simulink model "DMC_FCSMPC_IM_Physical_v6_3_L100_T1_EX28"  (R2021a)
settings: Solver=FixedStepDiscrete  StartTime=0.0  StopTime=3  FixedStep=1e-6  RelTol=1e-3
libraries: spsIGBTDiodeLib x18, spsCurrentMeasurementLib x3, spsThreePhaseSeriesRLCBranchLib x3, spsThreePhaseVIMeasurementLib x3, spsThreePhaseParallelRLCBranchLib x2, spsAsynchronousMachineSIUnitsLib x1, spsThreePhaseProgrammableVoltageSourceLib x1, spsGroundLib x1, spspowerguiLib x1
settings Model: Creator=edula  LastModifiedBy=Usuario

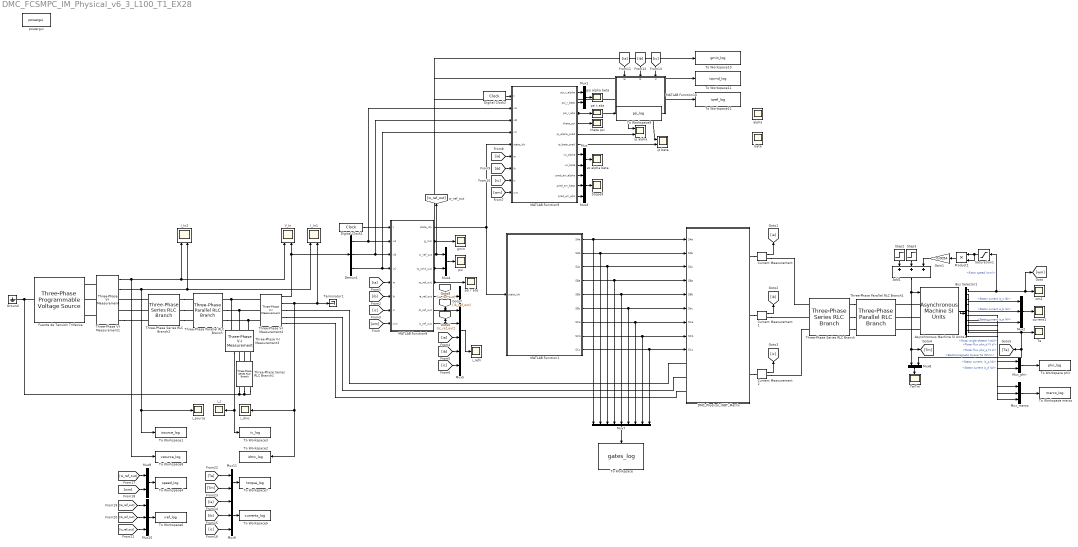
== system DMC_FCSMPC_IM_Physical_v6_3_L100_T1_EX28 ==
  Add1 : Sum  Inputs=+++
  Asynchronous Machine SI Units1 : spsAsynchronousMachineSIUnitsLib/Asynchronous Machine SI Units  RotorType=Squirrel-cage  PresetModel=No  MechanicalLoad=Torque Tm  ShowDetailedParameters=on  ReferenceFrame=Rotor  Units=SI  MeasurementBus=off  NominalParameters=[1.845e+04 380 50]  VoltageRatio=1  Stator=[0.5968 0.0003495]  Rotor=[0.6258 0.005473]  Cage1=[0.4155 0.002066]  Cage2=[0.4168 0.0003495]  Lm=0.0354  Mechanical=[0.08 0.005879 2]  PolePairs=2  InitialConditions=[1 0 0 0 0 0 0 0]  SimulateSaturation=off  Saturation=[14.03593122, 27.81365428, 53.79336849, 72.68890987, 97.98006896, 148.6815601, 215.7428561, 302.9841135, 428.7778367 ; 230, 322, 414, 460, 506, 552, 598, 644, 690]  LoadFlowParameters=1492000  TsPowergui=0  TsBlock=-1  IterativeModel=Trapezoidal non iterative  IterativeDiscreteModel=Trapezoidal non iterative  Pmec=1.492e+006
  Bus Selector1 : BusSelector  OutputSignals="Mechanical.Rotor speed (wm),Stator measurements.Stator current is_c (A),Stator measurements.Stator current is_b (A),Stator measurements.Stator current is_a (A),Mechanical.Electromagnetic torque Te (N*m),Rotor measurements.Rotor flux phir_q (V s),Rotor measurements.Rotor flux phir_d (V s),Mechanical.Rotor angle thetam (rad),Stator measurements.Stator current  is_q (A),Stator measurements.Stator current is_d (A)"
  Current Measurement : spsCurrentMeasurementLib/Current Measurement  PhasorSimulation=off  OutputType=Complex  PSBequivalent=0
  Current Measurement1 : spsCurrentMeasurementLib/Current Measurement  PhasorSimulation=off  OutputType=Complex  PSBequivalent=0
  Current Measurement2 : spsCurrentMeasurementLib/Current Measurement  PhasorSimulation=off  OutputType=Complex  PSBequivalent=0
  DMC_Physical_IGBT_Matrix : Subsystem
  Demux1 : Demux  Outputs=3
  Digital Clock1 : DigitalClock  SampleTime=1e-06
  Digital Clock2 : DigitalClock  SampleTime=1e-06
  Fuente de Tensión Trifásica : spsThreePhaseProgrammableVoltageSourceLib/Three-Phase Programmable Voltage Source  PositiveSequence=[380 0 50]  VariationEntity=Frequency  VariationType=Step  VariationTypeAlt=Ramp  VariationStep=0.5  VariationRate=0  VariationMagnitude=0.3  VariationFrequency=2  VariationTiming=[2 4]  VariationPhaseA=off  Amplitudes=[1 0.8 1.2 1.0]  TimeValues=[0 0.1 0.15 0.2]  HarmonicGeneration=off  HarmonicA=[3 0.2 -25 0]  HarmonicB=[2 0.15 35 2]  Timing="[0.05  3]"  BusType=swing  Pref=0  Qref=0  Qmin=-inf  Qmax=inf
  Gain1 : Gain  Gain=0.0054
  Ground : spsGroundLib/Ground  LConnTagsString=a
  I_In1 : Scope  NumInputPorts=2
  I_In2 : Scope  NumInputPorts=2
  MATLAB Function1 : MATLAB Function  TreatAsAtomicUnit=on
  MATLAB Function10 : MATLAB Function  TreatAsAtomicUnit=on
  MATLAB Function8 : MATLAB Function  TreatAsAtomicUnit=on
  MATLAB Function9 : MATLAB Function  TreatAsAtomicUnit=on
  Mux{,1,4,8..9,11} (6 alike) : Mux  Inputs=2
  Mux{2..3,6,10} (4 alike) : Mux  Inputs=3
  Mux5 : Mux  Inputs=6
  Mux7 : Mux  Inputs=9
  Mux_marco : Mux  Inputs=3
  Mux_phir : Mux  Inputs=2
  Product1 : Product  RndMeth=Zero
  Saturation1 : Saturate  UpperLimit=100000  LowerLimit=0
  Scope9 : Scope
  Step2 : Step  Time=0  After=0  SampleTime=0
  Step3 : Step  Time=0  After=5  SampleTime=0
  Te : Scope
  Te/Tm : Scope
  Terminator1 : Terminator
  Three-Phase Parallel RLC Branch : spsThreePhaseParallelRLCBranchLib/Three-Phase Parallel RLC Branch  LConnTagsString=A|B|C  RConnTagsString=A|B|C  BranchType=RL  Resistance=10  Inductance=0.0023  Capacitance=1.0  Measurements=None
      settings: SourceProductBaseCode=PS
  Three-Phase Parallel RLC Branch1 : spsThreePhaseParallelRLCBranchLib/Three-Phase Parallel RLC Branch  LConnTagsString=A|B|C  RConnTagsString=A|B|C  BranchType=RL  Resistance=25  Inductance=0.00000795  Capacitance=1e-6  Measurements=None
      settings: SourceProductBaseCode=PS
  Three-Phase Series RLC Branch : spsThreePhaseSeriesRLCBranchLib/Three-Phase Series RLC Branch  LConnTagsString=A|B|C  RConnTagsString=A|B|C  BranchType=R  Resistance=0.0525  Inductance=1e-3  Capacitance=1e-6  Measurements=None
  Three-Phase Series RLC Branch1 : spsThreePhaseSeriesRLCBranchLib/Three-Phase Series RLC Branch  LConnTagsString=A|B|C  RConnTagsString=A|B|C  BranchType=C  Resistance=1.0  Inductance=1.0  Capacitance=0.00001  Measurements=None
  Three-Phase Series RLC Branch2 : spsThreePhaseSeriesRLCBranchLib/Three-Phase Series RLC Branch  LConnTagsString=A|B|C  RConnTagsString=A|B|C  BranchType=RL  Resistance=0.0134  Inductance=0.0000259  Capacitance=1.0  Measurements=None
  Three-Phase V-I Measurement1 : spsThreePhaseVIMeasurementLib/Three-Phase V-I Measurement  VoltageMeasurement=phase-to-ground  SetLabelV=off  LabelV=Vabc  Vpu=off  VpuLL=off  CurrentMeasurement=yes  SetLabelI=off  LabelI=Iabc  Ipu=off  Pbase=100e6  Vbase=500e3  OutputType=Complex  PhasorSimulation=off  PSBequivalent=0
  Three-Phase V-I Measurement2 : spsThreePhaseVIMeasurementLib/Three-Phase V-I Measurement  VoltageMeasurement=phase-to-ground  SetLabelV=off  LabelV=Vabc  Vpu=off  VpuLL=off  CurrentMeasurement=yes  SetLabelI=off  LabelI=Iabc  Ipu=off  Pbase=100e6  Vbase=500e3  OutputType=Complex  PhasorSimulation=off  PSBequivalent=0
  Three-Phase V-I Measurement3 : spsThreePhaseVIMeasurementLib/Three-Phase V-I Measurement  VoltageMeasurement=phase-to-ground  SetLabelV=off  LabelV=Vabc  Vpu=off  VpuLL=off  CurrentMeasurement=yes  SetLabelI=off  LabelI=Iabc  Ipu=off  Pbase=100e6  Vbase=500e3  OutputType=Complex  PhasorSimulation=off  PSBequivalent=0
  To Workspace : ToWorkspace  VariableName=gates_log  SaveFormat=Structure With Time  SampleTime=-1
      settings: Decimation=200
  To Workspace marco : ToWorkspace  VariableName=marco_log  SaveFormat=Structure With Time  SampleTime=-1
      settings: Decimation=200
  To Workspace phir : ToWorkspace  VariableName=phir_log  SaveFormat=Structure With Time  SampleTime=-1
      settings: Decimation=200
  To Workspace1 : ToWorkspace  VariableName=isource_log  SaveFormat=Structure With Time  SampleTime=-1
      settings: Decimation=200
  To Workspace10 : ToWorkspace  VariableName=gmin_log  SaveFormat=Structure With Time  SampleTime=-1
      settings: Decimation=200
  To Workspace11 : ToWorkspace  VariableName=iqcmd_log  SaveFormat=Structure With Time  SampleTime=-1
      settings: Decimation=200
  To Workspace12 : ToWorkspace  VariableName=iqref_log  SaveFormat=Structure With Time  SampleTime=-1
      settings: Decimation=200
  To Workspace2 : ToWorkspace  VariableName=idmc_log  SaveFormat=Structure With Time  SampleTime=-1
      settings: Decimation=200
  To Workspace3 : ToWorkspace  VariableName=ic_log  SaveFormat=Structure With Time  SampleTime=-1
      settings: Decimation=200
  To Workspace4 : ToWorkspace  VariableName=speed_log  SaveFormat=Structure With Time  SampleTime=-1
      settings: Decimation=200
  To Workspace5 : ToWorkspace  VariableName=currents_log  SaveFormat=Structure With Time  SampleTime=-1
      settings: Decimation=200
  To Workspace6 : ToWorkspace  VariableName=iref_log  SaveFormat=Structure With Time  SampleTime=-1
      settings: Decimation=200
  To Workspace7 : ToWorkspace  VariableName=torque_log  SaveFormat=Structure With Time  SampleTime=-1
      settings: Decimation=200
  To Workspace8 : ToWorkspace  VariableName=vsource_log  SaveFormat=Structure With Time  SampleTime=-1
      settings: Decimation=200
  To Workspace9 : ToWorkspace  VariableName=psi_log  SaveFormat=Structure With Time  SampleTime=-1
      settings: Decimation=200
  V_In : Scope  NumInputPorts=2
  alpha : Scope  NumInputPorts=2
  beta : Scope  NumInputPorts=2
  current1 : Scope
  gmin : Scope
  i_c : Scope
  i_dmc : Scope
  i_ref/i : Scope
  i_source : Scope
  ip alpha : Scope  NumInputPorts=2
  ip beta : Scope  NumInputPorts=2
  powergui : spspowerguiLib/powergui  Priority=1  SimulationMode=Discrete  SampleTime=1e-6  frequency=60  Iterations=50  frequencyindice=50  Pbase=100e6  ErrMax=1e-4  UnitsV=kV  UnitsW=MW  buscounter=0  FunctionMessages=off  echomessages=off  EnableUseOfTLC=off  CurrentSourceSwitches=off  DisableSnubberDevices=off  DisableRonSwitches=off  DisableVfSwitches=off  DisplayEquations=off  AutomaticDiscreteSolvers=off  SolverType=Tustin/Backward Euler (TBE)  Interpol=off  ExternalGateDelay=off  methode=off  Ts=100  x0status=blocks  SPID=on  SwTol=0  HookPort=off  NonlinearTolerance=1e-4  nMaxIteration=100  ContinueOnMaxIteration=off  RestoreLinks=warning  ResistiveCurrentMeasurement=off  Frange=[0:2:500]  Ylog=off  Xlog=on  ShowGrid=off  save=off  variable=ZData  structure=0  ZoomFFT=off  StartTime=0.0  cycles=1  DisplayStyle=1  fundamental=60  FreqAxis=off  MaxFrequency=1000  frequencyindicesteady=1  RmsSteady=1  display=off
  psi : Scope
  psi alpha beta : Scope
  psi r abs : Scope
  psi t abs : Scope
  theta psi : Scope
  vo alpha beta : Scope
  wm1 : Scope
  wires:
  Product1/1 -> Gain1/1
  Gain1/1 -> Add1/3
  Step3/1 -> Add1/2
  Mux2/1 -> current1/1
  Bus Selector1/1 -> [wm], wm1/1, Saturation1/1  "<Rotor speed (wm)>"
  Bus Selector1/3 -> Mux2/2  "<Stator current is_b (A)>"
  Bus Selector1/2 -> Mux2/1  "<Stator current is_c (A)>"
  Saturation1/1 -> Product1/1, Product1/2
  Bus Selector1/4 -> Mux2/3  "<Stator current is_a (A)>"
  Step2/1 -> Add1/1
  Asynchronous Machine SI Units1/1 -> Bus Selector1/1
  Demux1/1 -> MATLAB Function8/2(vA), MATLAB Function9/2(vA)
  Demux1/3 -> MATLAB Function9/4(vC), MATLAB Function8/4(vC)
  Demux1/2 -> MATLAB Function9/3(vB), MATLAB Function8/3(vB)
  Three-Phase V-I Measurement2/1 -> V_In/2, Demux1/1
  Digital Clock1/1 -> MATLAB Function8/1(t)
  Current Measurement/1 -> [ia]
  Current Measurement1/1 -> [ib]
  Current Measurement2/1 -> [ic]
  MATLAB Function8/1(state_idx) -> MATLAB Function9/5(state_idx), MATLAB Function1/1(state_idx)
  [wm] -> MATLAB Function8/8(wm)
  [ic] -> MATLAB Function8/7(ic)
  [ia] -> MATLAB Function8/5(ia)
  [ib] -> MATLAB Function8/6(ib)
  MATLAB Function8/2(g_min) -> gmin/1, To Workspace10/1
  [wm] -> MATLAB Function9/9(wm)
  [ia] -> MATLAB Function9/6(ia)
  [ib] -> MATLAB Function9/7(ib)
  [ic] -> MATLAB Function9/8(ic)
  MATLAB Function9/4(theta_psi) -> theta psi/1
  MATLAB Function9/3(psi_r_abs) -> psi t abs/1, To Workspace9/1
  MATLAB Function9/6(ip_beta_pred) -> ip beta/2
  [ic] -> MATLAB Function10/3(ic)
  MATLAB Function10/2(i_beta) -> ip beta/1
  MATLAB Function8/5(iq_ref_out) -> psi r abs/1, To Workspace12/1
  MATLAB Function1/1(SAa) -> Mux7/1, DMC_Physical_IGBT_Matrix/1(SAa)
  MATLAB Function1/2(SAb) -> Mux7/2, DMC_Physical_IGBT_Matrix/2(SAb)
  MATLAB Function1/3(SAc) -> Mux7/3, DMC_Physical_IGBT_Matrix/3(SAc)
  MATLAB Function1/4(SBa) -> Mux7/4, DMC_Physical_IGBT_Matrix/4("SBa\t\t")
  MATLAB Function1/5(SBb) -> DMC_Physical_IGBT_Matrix/5(SBb), Mux7/5
  MATLAB Function1/6(SBc) -> Mux7/6, DMC_Physical_IGBT_Matrix/6(Sbc)
  MATLAB Function1/7(SCa) -> DMC_Physical_IGBT_Matrix/7(SCa), Mux7/7
  MATLAB Function1/8(SCb) -> Mux7/8, DMC_Physical_IGBT_Matrix/8(SCb)
  MATLAB Function1/9(SCc) -> DMC_Physical_IGBT_Matrix/9(SCc), Mux7/9
  Digital Clock2/1 -> MATLAB Function9/1(t)
  [ia] -> MATLAB Function10/1(ia)
  [ib] -> MATLAB Function10/2(ib)
  MATLAB Function9/7(vo_alpha) -> Mux/1
  MATLAB Function9/8(vo_beta) -> Mux/2
  Mux/1 -> vo alpha beta/1
  MATLAB Function9/1(psi_r_alpha) -> Mux1/1
  MATLAB Function9/2(psi_r_beta) -> Mux1/2
  Mux1/1 -> psi alpha beta/1
  MATLAB Function9/9(pred_err_alpha) -> Mux3/1
  MATLAB Function9/10(pred_err_beta) -> Mux3/2
  MATLAB Function9/11(pred_err_abs) -> Mux3/3
  Mux3/1 -> Scope9/1
  MATLAB Function8/3(w_ref_out) -> Mux4/1, [w_ref_out]
  MATLAB Function8/4(iq_cmd_out) -> Mux4/2, To Workspace11/1
  Mux4/1 -> psi/1
  MATLAB Function8/6(ia_ref_out) -> [ia_ref_out], Mux5/1
  MATLAB Function8/7(ib_ref_out) -> [ib_ref_out], Mux5/2
  MATLAB Function8/8(ic_ref_out) -> [ic_ref_out], Mux5/3
  Mux5/1 -> i_ref/i/1
  [ia] -> Mux5/4
  [ib] -> Mux5/5
  [ic] -> Mux5/6
  Three-Phase V-I Measurement1/1 -> To Workspace8/1, I_In2/1, V_In/1
  Three-Phase V-I Measurement1/2 -> I_In1/1, I_In2/2, To Workspace1/1, i_source/1
  Three-Phase V-I Measurement2/2 -> Terminator1/1, I_In1/2, To Workspace2/1, i_dmc/1
  MATLAB Function10/1(i_alpha) -> ip alpha/1
  MATLAB Function9/5(ip_alpha_pred) -> ip alpha/2
  Add1/1 -> Mux8/1, [Tm], Asynchronous Machine SI Units1/1
  Bus Selector1/5 -> Mux8/2, [Te], Te/1  "<Electromagnetic torque Te (N*m)>"
  Mux8/1 -> Te/Tm/1
  Three-Phase V-I Measurement3/2 -> i_c/1, To Workspace3/1
  Mux6/1 -> To Workspace5/1
  [ia] -> Mux6/1
  [ib] -> Mux6/2
  [ic] -> Mux6/3
  Mux7/1 -> To Workspace/1
  [w_ref_out] -> Mux9/1
  [wm] -> Mux9/2
  Mux9/1 -> To Workspace4/1
  [ia_ref_out] -> Mux10/1
  [ib_ref_out] -> Mux10/2
  [ic_ref_out] -> Mux10/3
  Mux10/1 -> To Workspace6/1
  [Te] -> Mux11/1
  [Tm] -> Mux11/2
  Mux11/1 -> To Workspace7/1
  Bus Selector1/6 -> Mux_phir/1  "<Rotor flux phir_q (V s)>"
  Bus Selector1/7 -> Mux_phir/2  "<Rotor flux phir_d (V s)>"
  Bus Selector1/8 -> Mux_marco/1  "<Rotor angle thetam (rad)>"
  Bus Selector1/9 -> Mux_marco/2  "<Stator current  is_q (A)>"
  Bus Selector1/10 -> Mux_marco/3  "<Stator current is_d (A)>"
  Mux_phir/1 -> To Workspace phir/1
  Mux_marco/1 -> To Workspace marco/1
  connections:
  DMC_Physical_IGBT_Matrix/RConn1 -- Current Measurement/LConn1
  DMC_Physical_IGBT_Matrix/RConn2 -- Current Measurement1/LConn1
  DMC_Physical_IGBT_Matrix/RConn3 -- Current Measurement2/LConn1
  Three-Phase V-I Measurement2/RConn1 -- DMC_Physical_IGBT_Matrix/LConn1
  Three-Phase V-I Measurement2/RConn2 -- DMC_Physical_IGBT_Matrix/LConn2
  Three-Phase V-I Measurement2/RConn3 -- DMC_Physical_IGBT_Matrix/LConn3
  Three-Phase Parallel RLC Branch/RConn3 -- Three-Phase V-I Measurement2/LConn3 -- Three-Phase V-I Measurement3/LConn3
  Three-Phase V-I Measurement2/LConn1 -- Three-Phase V-I Measurement3/LConn1 -- Three-Phase Parallel RLC Branch/RConn1
  Three-Phase Series RLC Branch1/RConn2 -- Three-Phase Series RLC Branch1/RConn3 -- Fuente de Tensión Trifásica/LConn1 -- Ground/LConn1 -- Three-Phase Series RLC Branch1/RConn1
  Three-Phase Parallel RLC Branch/RConn2 -- Three-Phase V-I Measurement2/LConn2 -- Three-Phase V-I Measurement3/LConn2
  Three-Phase V-I Measurement1/LConn1 -- Fuente de Tensión Trifásica/RConn1
  Three-Phase V-I Measurement1/LConn2 -- Fuente de Tensión Trifásica/RConn2
  Three-Phase V-I Measurement1/LConn3 -- Fuente de Tensión Trifásica/RConn3
  Three-Phase Series RLC Branch2/RConn1 -- Three-Phase Parallel RLC Branch/LConn1
  Three-Phase Series RLC Branch2/RConn2 -- Three-Phase Parallel RLC Branch/LConn2
  Three-Phase Series RLC Branch2/RConn3 -- Three-Phase Parallel RLC Branch/LConn3
  Asynchronous Machine SI Units1/LConn2 -- Three-Phase Parallel RLC Branch1/RConn2
  Asynchronous Machine SI Units1/LConn3 -- Three-Phase Parallel RLC Branch1/RConn3
  Asynchronous Machine SI Units1/LConn1 -- Three-Phase Parallel RLC Branch1/RConn1
  Current Measurement2/RConn1 -- Three-Phase Series RLC Branch/LConn3
  Current Measurement1/RConn1 -- Three-Phase Series RLC Branch/LConn2
  Current Measurement/RConn1 -- Three-Phase Series RLC Branch/LConn1
  Three-Phase Series RLC Branch2/LConn1 -- Three-Phase V-I Measurement1/RConn1
  Three-Phase Series RLC Branch2/LConn2 -- Three-Phase V-I Measurement1/RConn2
  Three-Phase V-I Measurement1/RConn3 -- Three-Phase Series RLC Branch2/LConn3
  Three-Phase Series RLC Branch1/LConn1 -- Three-Phase V-I Measurement3/RConn1
  Three-Phase Series RLC Branch1/LConn2 -- Three-Phase V-I Measurement3/RConn2
  Three-Phase Series RLC Branch1/LConn3 -- Three-Phase V-I Measurement3/RConn3
  Three-Phase Series RLC Branch/RConn1 -- Three-Phase Parallel RLC Branch1/LConn1
  Three-Phase Series RLC Branch/RConn2 -- Three-Phase Parallel RLC Branch1/LConn2
  Three-Phase Series RLC Branch/RConn3 -- Three-Phase Parallel RLC Branch1/LConn3

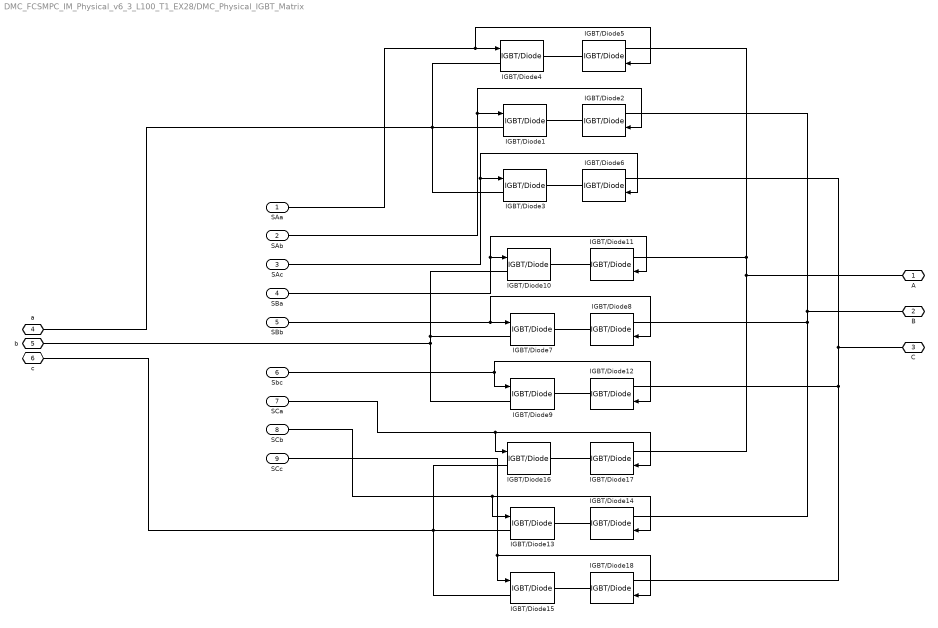
== system DMC_FCSMPC_IM_Physical_v6_3_L100_T1_EX28/DMC_Physical_IGBT_Matrix ==
  SAa : Inport
  SAb : Inport  Port=2
  SAc : Inport  Port=3
  "SBa\t\t" : Inport  Port=4
  SBb : Inport  Port=5
  Sbc : Inport  Port=6
  SCa : Inport  Port=7
  SCb : Inport  Port=8
  SCc : Inport  Port=9
  IGBT/Diode{1,3..4,7,9..10,13,15..16} (9 alike) : spsIGBTDiodeLib/IGBT//Diode  Ron=0.01  Rs=1e5  Cs=1e-9  Measurements=off
  IGBT/Diode{2,5..6,8,11..12,14,17..18} (9 alike) : spsIGBTDiodeLib/IGBT//Diode  Ron=1e-3  Rs=1e5  Cs=1e-9  Measurements=off
  A : PMIOPort  Side=Right
  B : PMIOPort  Port=2  Side=Right
  C : PMIOPort  Port=3  Side=Right
  a : PMIOPort  Port=4  Side=Left
  b : PMIOPort  Port=5  Side=Left
  c : PMIOPort  Port=6  Side=Left
  wires:
  SCc/1 -> IGBT/Diode15/1, IGBT/Diode18/1
  Sbc/1 -> IGBT/Diode12/1, IGBT/Diode9/1
  SAc/1 -> IGBT/Diode6/1, IGBT/Diode3/1
  SAb/1 -> IGBT/Diode2/1, IGBT/Diode1/1
  SAa/1 -> IGBT/Diode5/1, IGBT/Diode4/1
  SBb/1 -> IGBT/Diode8/1, IGBT/Diode7/1
  "SBa\t\t"/1 -> IGBT/Diode11/1, IGBT/Diode10/1
  SCb/1 -> IGBT/Diode13/1, IGBT/Diode14/1
  SCa/1 -> IGBT/Diode16/1, IGBT/Diode17/1
  connections:
  IGBT/Diode3/RConn1 -- IGBT/Diode6/RConn1
  IGBT/Diode8/LConn1 -- IGBT/Diode14/LConn1 -- B/RConn1 -- IGBT/Diode2/LConn1
  IGBT/Diode9/RConn1 -- IGBT/Diode12/RConn1
  IGBT/Diode5/LConn1 -- A/RConn1 -- IGBT/Diode17/LConn1 -- IGBT/Diode11/LConn1
  IGBT/Diode13/RConn1 -- IGBT/Diode14/RConn1
  IGBT/Diode10/RConn1 -- IGBT/Diode11/RConn1
  IGBT/Diode9/LConn1 -- IGBT/Diode7/LConn1 -- IGBT/Diode10/LConn1 -- b/RConn1
  IGBT/Diode15/RConn1 -- IGBT/Diode18/RConn1
  IGBT/Diode18/LConn1 -- IGBT/Diode12/LConn1 -- C/RConn1 -- IGBT/Diode6/LConn1
  IGBT/Diode16/LConn1 -- c/RConn1 -- IGBT/Diode13/LConn1 -- IGBT/Diode15/LConn1
  IGBT/Diode1/RConn1 -- IGBT/Diode2/RConn1
  IGBT/Diode16/RConn1 -- IGBT/Diode17/RConn1
  IGBT/Diode7/RConn1 -- IGBT/Diode8/RConn1
  IGBT/Diode3/LConn1 -- a/RConn1 -- IGBT/Diode4/LConn1 -- IGBT/Diode1/LConn1
  IGBT/Diode4/RConn1 -- IGBT/Diode5/RConn1

== matlab function DMC_FCSMPC_IM_Physical_v6_3_L100_T1_EX28/MATLAB Function1 ==
  data: state_idx input; SAa output; SAb output; SAc output; SBa output; SBb output; SBc output; SCa output; SCb output; SCc output
function [SAa,SAb,SAc,SBa,SBb,SBc,SCa,SCb,SCc] = DMC_StateToGates(state_idx)
%#codegen
% DMC state decoder.
%
% state_idx selects one of 27 valid DMC states.
%
% Signal naming:
% Sxy = input phase x connected to output phase y
%
% Inputs:
%   A = 1
%   B = 2
%   C = 3
%
% sel_a = selected input connected to motor phase a
% sel_b = selected input connected to motor phase b
% sel_c = selected input connected to motor phase c

    idx = round(state_idx);

    if idx < 1 || idx > 27
        idx = 1;
    end

    % First states are placed manually for easy testing.
    %
    % 1: A->a, B->b, C->c  pass-through
    % 2: C->a, A->b, B->c  cyclic permutation
    % 3: B->a, C->b, A->c  cyclic permutation
    % 4: A->a, C->b, B->c  reversed sequence
    % 5: B->a, A->b, C->c  reversed sequence
    % 6: C->a, B->b, A->c  reversed sequence
    %
    % Remaining states complete the 27 possible combinations.

    sel_a = [ ...
        1 3 2 1 2 3 ...
        1 1 1 1 1 1 1 ...
        2 2 2 2 2 2 2 ...
        3 3 3 3 3 3 3 ];

    sel_b = [ ...
        2 1 3 3 1 2 ...
        1 1 1 2 2 3 3 ...
        1 1 2 2 2 3 3 ...
        1 1 2 2 3 3 3 ];

    sel_c = [ ...
        3 2 1 2 3 1 ...
        1 2 3 1 2 1 3 ...
        1 2 1 2 3 2 3 ...
        1 3 2 3 1 2 3 ];

    ia = sel_a(idx);
    ib = sel_b(idx);
    ic = sel_c(idx);

    % Output phase a
    SAa = double(ia == 1);
    SBa = double(ia == 2);
    SCa = double(ia == 3);

    % Output phase b
    SAb = double(ib == 1);
    SBb = double(ib == 2);
    SCb = double(ib == 3);

    % Output phase c
    SAc = double(ic == 1);
    SBc = double(ic == 2);
    SCc = double(ic == 3);
end

== matlab function DMC_FCSMPC_IM_Physical_v6_3_L100_T1_EX28/MATLAB Function8 ==
  data: t input; state_idx output; vA input; vB input; vC input; ia input; ib input; ic input; wm input; g_min output; w_ref_out output; iq_cmd_out output; iq_ref_out output; ia_ref_out output; ib_ref_out output; ic_ref_out output
function [state_idx, g_min, w_ref_out, iq_cmd_out, iq_ref_out,ia_ref_out, ib_ref_out, ic_ref_out] = fcn(t,vA,vB,vC,ia,ib,ic,wm)
%#codegen
%
% FCS-MPC de corriente para DMC fisico + motor de induccion.
%
% Version limpia:
%   1) Sin arranque auxiliar por tension.
%   2) Referencia de velocidad rampada.
%   3) Estimador interno de flujo rotorico.
%   4) Referencia de corriente orientada por flujo: id / iq.
%   5) Lazo externo proporcional de velocidad.
%   6) Filtro suave de iq para reducir cambios bruscos de torque.
%   7) Busqueda exhaustiva sobre estados finitos del DMC.
%
% Entradas:
%   t          tiempo [s]
%   vA,vB,vC  tensiones de entrada reales del DMC [V]
%   ia,ib,ic  corrientes medidas entre DMC y motor [A]
%   wm         velocidad mecanica del rotor [rad/s]
%
% Salidas:
%   state_idx     indice de estado para DMC_StateToGates
%   g_min         costo minimo encontrado
%   ia_ref_out    referencia corriente fase a [A]
%   ib_ref_out    referencia corriente fase b [A]
%   ic_ref_out    referencia corriente fase c [A]
%   w_ref_out     referencia de velocidad rampada [rad/s]
%   iq_cmd_out    comando instantaneo de corriente de torque [A]
%   iq_ref_out    referencia de corriente q filtrada y usada [A]

    % ==============================================================
    % 1) Parametros generales de control
    % ==============================================================

    Ts_ctrl = 2e-4;          % [s] periodo de control, 5 kHz

    lambda_sw = 100;       % penalizacion de conmutacion
    Imax = 300.0;            % [A] limite defensivo de corriente predicha

    % Referencias base en dq
    id_ref_final = 28.0;     % [A] corriente de magnetizacion / flujo
    iq_sign = 1.0;           % signo validado para producir torque positivo

    % Referencia de velocidad
    w_ref_final = 95.0;      % [rad/s] velocidad objetivo final
    w_ramp_time = 1.0;       % [s] tiempo para llevar w_ref de 0 a w_ref_final

    % Lazo externo de velocidad
    Kp_w = 20.0; %tenia 10            % ganancia proporcional de velocidad

    % Limites de corriente q
    iq_min = 0.0;            % [A]
    iq_max = 50.0;           % [A]

    % Filtro de iq
    alpha_iq = 0.05;         % 0 < alpha_iq <= 1

    % Angulo auxiliar si el flujo estimado todavia es bajo
    f_fallback = 30.0;       % [Hz]

    % ==============================================================
    % 2) Parametros del motor de induccion
    % ==============================================================

    Rs  = 0.5968;            % [ohm]
    Lls = 0.0003495;         % [H]

    Rr  = 0.6258;            % [ohm] referido al estator
    Llr = 0.005473;          % [H]

    Lm  = 0.0354;            % [H]

    p = 2.0;                 % pares de polos

    Ls = Lls + Lm;
    Lr = Llr + Lm;

    sigma = 1.0 - (Lm*Lm)/(Ls*Lr);
    kr = Lm/Lr;

    R_sigma = Rs + Rr*kr*kr;

    tau_r = Lr/Rr;
    tau_sigma = sigma*Ls/R_sigma;

    omega_r = p*wm;

    % ==============================================================
    % 3) Variables persistentes
    % ==============================================================

    persistent last_idx last_k
    persistent psi_a psi_b
    persistent g_last
    persistent ia_ref_last ib_ref_last ic_ref_last
    persistent w_ref_last iq_cmd_last iq_ref_last
    persistent iq_cmd_f

    if isempty(last_idx)
        last_idx = 1;
        last_k = -1;

        psi_a = 0.0;
        psi_b = 0.0;

        g_last = 0.0;

        ia_ref_last = 0.0;
        ib_ref_last = 0.0;
        ic_ref_last = 0.0;

        w_ref_last = 0.0;
        iq_cmd_last = 0.0;
        iq_ref_last = 0.0;

        iq_cmd_f = 0.0;
    end

    k = floor(t/Ts_ctrl);

    % Mantener el estado y las salidas durante el mismo intervalo de control.
    if k == last_k
        state_idx = last_idx;
        g_min = g_last;

        ia_ref_out = ia_ref_last;
        ib_ref_out = ib_ref_last;
        ic_ref_out = ic_ref_last;

        w_ref_out = w_ref_last;
        iq_cmd_out = iq_cmd_last;
        iq_ref_out = iq_ref_last;

        return;
    end

    last_k = k;

    % ==============================================================
    % 4) Corrientes medidas abc -> alpha-beta
    % ==============================================================

    i_alpha = (2.0/3.0)*(ia - 0.5*ib - 0.5*ic);
    i_beta  = (1.0/sqrt(3.0))*(ib - ic);

    % ==============================================================
    % 5) Estimador interno de flujo rotorico
    % ==============================================================
    %
    % Modelo en marco estacionario alpha-beta:
    %
    % dpsi_alpha = (-psi_alpha + Lm*i_alpha)/tau_r - omega_r*psi_beta
    % dpsi_beta  = (-psi_beta  + Lm*i_beta )/tau_r + omega_r*psi_alpha

    % Discretizacion exacta (ZOH sobre i), no Euler explicito:
    %   psi(k+1) = Phi*psi(k) + G*Lm*i(k)
    %   Phi = exp(A*Ts),  G = (Phi-1)/(A*tau_r),  A = -1/tau_r + j*omega_r
    ea = exp(-Ts_ctrl/tau_r);
    Phi_re = ea*cos(omega_r*Ts_ctrl);
    Phi_im = ea*sin(omega_r*Ts_ctrl);
    den_A = (1.0/tau_r)^2 + omega_r^2;
    G_re = (-(Phi_re - 1.0)/tau_r + Phi_im*omega_r)/(den_A*tau_r);
    G_im = (-Phi_im/tau_r - (Phi_re - 1.0)*omega_r)/(den_A*tau_r);

    psi_a_next = Phi_re*psi_a - Phi_im*psi_b + Lm*(G_re*i_alpha - G_im*i_beta);
    psi_b_next = Phi_im*psi_a + Phi_re*psi_b + Lm*(G_im*i_alpha + G_re*i_beta);

    if ~isfinite(psi_a_next)
        psi_a_next = 0.0;
    end

    if ~isfinite(psi_b_next)
        psi_b_next = 0.0;
    end

    psi_a = psi_a_next;
    psi_b = psi_b_next;

    psi_abs_now = sqrt(psi_a*psi_a + psi_b*psi_b);

    % ==============================================================
    % 6) Referencia de velocidad rampada
    % ==============================================================

    w_ramp = t / w_ramp_time;

    if w_ramp > 1.0
        w_ramp = 1.0;
    elseif w_ramp < 0.0
        w_ramp = 0.0;
    end

    w_ref = w_ref_final * w_ramp;

    % ==============================================================
    % 7) Lazo externo de velocidad
    % ==============================================================

    speed_err = w_ref - wm;

    iq_cmd = Kp_w * speed_err;

    if iq_cmd > iq_max
        iq_cmd = iq_max;
    elseif iq_cmd < iq_min
        iq_cmd = iq_min;
    end

    % Filtro discreto de primer orden:
    % iq_cmd_f(k) = iq_cmd_f(k-1) + alpha_iq*(iq_cmd - iq_cmd_f(k-1))
    iq_cmd_f = iq_cmd_f + alpha_iq*(iq_cmd - iq_cmd_f);

    if iq_cmd_f > iq_max
        iq_cmd_f = iq_max;
    elseif iq_cmd_f < iq_min
        iq_cmd_f = iq_min;
    end

    id_ref = id_ref_final;
    iq_ref = iq_sign * iq_cmd_f;

    % ==============================================================
    % 8) Orientacion por flujo y referencia de corriente
    % ==============================================================

    % Si el flujo es muy bajo, atan2 no es confiable.
    % En ese caso se usa un angulo auxiliar giratorio.
    psi_min = 0.05;

    if psi_abs_now > psi_min
        theta_psi = atan2(psi_b, psi_a);
        % ADELANTO DE UN PASO (variante T1 del experimento).
        % El MPC compara i_ref(k) contra la corriente predicha en k+1, asi
        % que la referencia tiene que generarse con el angulo que el flujo
        % va a tener en k+1, no con el de k.
        w_slip_est = Lm*iq_ref/(tau_r*psi_abs_now);
        theta_psi = theta_psi + (omega_r + w_slip_est)*Ts_ctrl;
    else
        theta_psi = 2.0*pi*f_fallback*t;
    end

    cth = cos(theta_psi);
    sth = sin(theta_psi);

    % Inversa dq -> alpha-beta, con eje d alineado al flujo rotorico.
    iref_alpha = id_ref*cth - iq_ref*sth;
    iref_beta  = id_ref*sth + iq_ref*cth;

    % alpha-beta -> abc para monitoreo.
    ia_ref = iref_alpha;
    ib_ref = -0.5*iref_alpha + (sqrt(3.0)/2.0)*iref_beta;
    ic_ref = -0.5*iref_alpha - (sqrt(3.0)/2.0)*iref_beta;

    ia_ref_last = ia_ref;
    ib_ref_last = ib_ref;
    ic_ref_last = ic_ref;

    w_ref_last = w_ref;
    iq_cmd_last = iq_cmd;
    iq_ref_last = iq_ref;

    % ==============================================================
    % 9) Tabla de estados del DMC
    % ==============================================================
    %
    % Cada estado idx define de que fase de entrada se alimenta cada
    % fase de salida del DMC:
    %
    %   src_a = sel_a(idx)
    %   src_b = sel_b(idx)
    %   src_c = sel_c(idx)

    sel_a = [ ...
        1 3 2 1 2 3 ...
        1 1 1 1 1 1 1 ...
        2 2 2 2 2 2 2 ...
        3 3 3 3 3 3 3 ];

    sel_b = [ ...
        2 1 3 3 1 2 ...
        1 1 1 2 2 3 3 ...
        1 1 2 2 2 3 3 ...
        1 1 2 2 3 3 3 ];

    sel_c = [ ...
        3 2 1 2 3 1 ...
        1 2 3 1 2 1 3 ...
        1 2 1 2 3 2 3 ...
        1 3 2 3 1 2 3 ];

    % Estados cero excluidos:
    %   7  = A A A
    %   17 = B B B
    %   27 = C C C
    candidate_states = [ ...
        1 2 3 4 5 6 ...
        8 9 10 11 12 13 14 ...
        15 16 18 19 20 21 ...
        22 23 24 25 26 ];

    vin = [vA vB vC];

    ia_prev = sel_a(last_idx);
    ib_prev = sel_b(last_idx);
    ic_prev = sel_c(last_idx);

    best_idx = last_idx;
    best_cost = 1.0e30;

    % ==============================================================
    % 10) Busqueda exhaustiva FCS-MPC
    % ==============================================================

    for kk = 1:length(candidate_states)

        idx = candidate_states(kk);

        src_a = sel_a(idx);
        src_b = sel_b(idx);
        src_c = sel_c(idx);

        % ----------------------------------------------------------
        % 10.1) Tension de salida candidata
        % ----------------------------------------------------------

        vo_a = vin(src_a);
        vo_b = vin(src_b);
        vo_c = vin(src_c);

        vo_alpha = (2.0/3.0)*(vo_a - 0.5*vo_b - 0.5*vo_c);
        vo_beta  = (1.0/sqrt(3.0))*(vo_b - vo_c);

        % ----------------------------------------------------------
        % 10.2) Predictor de corriente de maquina de induccion
        % ----------------------------------------------------------

        aux_a = psi_a/tau_r + omega_r*psi_b;
        aux_b = psi_b/tau_r - omega_r*psi_a;

        di_a = ( -i_alpha + (kr/R_sigma)*aux_a + vo_alpha/R_sigma )/tau_sigma;
        di_b = ( -i_beta  + (kr/R_sigma)*aux_b + vo_beta /R_sigma )/tau_sigma;

        ip_alpha = i_alpha + Ts_ctrl*di_a;
        ip_beta  = i_beta  + Ts_ctrl*di_b;

        % ----------------------------------------------------------
        % 10.3) Costo de seguimiento de corriente
        % ----------------------------------------------------------

        err_alpha = iref_alpha - ip_alpha;
        err_beta  = iref_beta  - ip_beta;

        Ji = err_alpha*err_alpha + err_beta*err_beta;

        % ----------------------------------------------------------
        % 10.4) Penalizacion de conmutacion
        % ----------------------------------------------------------

        Nsw = 0.0;

        if src_a ~= ia_prev
            Nsw = Nsw + 1.0;
        end

        if src_b ~= ib_prev
            Nsw = Nsw + 1.0;
        end

        if src_c ~= ic_prev
            Nsw = Nsw + 1.0;
        end

        Jsw = lambda_sw*Nsw;

        % ----------------------------------------------------------
        % 10.5) Limite defensivo de corriente predicha
        % ----------------------------------------------------------

        ip_abs = sqrt(ip_alpha*ip_alpha + ip_beta*ip_beta);

        if ip_abs > Imax
            Jlim = 1.0e20;
        else
            Jlim = 0.0;
        end

        % ----------------------------------------------------------
        % 10.6) Costo total
        % ----------------------------------------------------------

        cost = Ji + Jsw + Jlim;

        if cost < best_cost
            best_cost = cost;
            best_idx = idx;
        end
    end

    % ==============================================================
    % 11) Salidas
    % ==============================================================

    last_idx = best_idx;
    g_last = best_cost;

    state_idx = last_idx;
    g_min = best_cost;

    ia_ref_out = ia_ref;
    ib_ref_out = ib_ref;
    ic_ref_out = ic_ref;

    w_ref_out = w_ref;
    iq_cmd_out = iq_cmd;
    iq_ref_out = iq_ref;
end

== matlab function DMC_FCSMPC_IM_Physical_v6_3_L100_T1_EX28/MATLAB Function9 ==
  data: t input; psi_r_alpha output; vA input; vB input; vC input; state_idx input; ia input; ib input; ic input; wm input; psi_r_beta output; psi_r_abs output; theta_psi output; ip_alpha_pred output; ip_beta_pred output; vo_alpha output; vo_beta output; pred_err_alpha output; pred_err_beta output; pred_err_abs output
function [psi_r_alpha, psi_r_beta, psi_r_abs, theta_psi, ip_alpha_pred, ip_beta_pred, vo_alpha, vo_beta, pred_err_alpha, pred_err_beta, pred_err_abs] = IM_FluxEstimator_Monitor(t, vA, vB, vC, state_idx, ia, ib, ic, wm)%#codegen
% IM_FluxEstimator_Monitor
%
% Estimador/monitor de flujo rotorico para maquina de induccion alimentada
% por DMC fisico.
%
% Este bloque NO controla el DMC.
% Este bloque NO genera state_idx.
% Este bloque solo estima psi_r y predice una muestra de corriente para
% validar el modelo antes de usarlo dentro del MPC.
%
% Entradas:
%   t         tiempo [s]
%   vA,vB,vC  tensiones de entrada al DMC [V]
%   state_idx estado aplicado por el selector/DMC_StateToGates [1..27]
%   ia,ib,ic  corrientes medidas entre DMC y motor [A]
%   wm        velocidad mecanica del rotor [rad/s]
%
% Salidas:
%   psi_r_alpha, psi_r_beta : flujo rotorico estimado en alpha-beta [Wb]
%   psi_r_abs              : modulo del flujo rotorico [Wb]
%   theta_psi              : angulo del flujo rotorico [rad]
%   ip_alpha_pred/ip_beta_pred : corriente predicha una muestra adelante [A]
%   vo_alpha/vo_beta       : tension alpha-beta aplicada reconstruida [V]

    % ==============================================================
    % 1) Tiempo de actualizacion
    % ==============================================================

    Ts_ctrl = 2e-4;   % [s] igual al selector actual

    persistent last_k
    persistent psi_a psi_b
    persistent ip_a_out ip_b_out
    persistent vo_a_out vo_b_out
    persistent ip_a_prev ip_b_prev
    persistent err_a_out err_b_out err_abs_out
    persistent pred_valid

    if isempty(last_k)
        last_k = -1;
        psi_a = 0.0;
        psi_b = 0.0;
        ip_a_out = 0.0;
        ip_b_out = 0.0;
        vo_a_out = 0.0;
        vo_b_out = 0.0;

        ip_a_prev = 0.0;
        ip_b_prev = 0.0;

        err_a_out = 0.0;
        err_b_out = 0.0;
        err_abs_out = 0.0;

        pred_valid = false;
    end

    k = floor(t/Ts_ctrl);

    % Si Simulink llama varias veces dentro del mismo periodo de control,
    % mantener la salida anterior.
    if k == last_k
        psi_r_alpha  = psi_a;
        psi_r_beta   = psi_b;
        psi_r_abs    = sqrt(psi_a*psi_a + psi_b*psi_b);
        theta_psi    = atan2(psi_b, psi_a);

        ip_alpha_pred = ip_a_out;
        ip_beta_pred  = ip_b_out;

        vo_alpha = vo_a_out;
        vo_beta  = vo_b_out;

        pred_err_alpha = err_a_out;
        pred_err_beta  = err_b_out;
        pred_err_abs   = err_abs_out;

        return;
    end

    last_k = k;

    % ==============================================================
    % 2) Parametros del motor
    % ==============================================================

    Rs  = 0.5968;       % [ohm]
    Lls = 0.0003495;    % [H]

    Rr  = 0.6258;       % [ohm] referido al estator
    Llr = 0.005473;     % [H] referido al estator

    Lm  = 0.0354;       % [H]

    p   = 2.0;          % pares de polos

    Ls = Lls + Lm;
    Lr = Llr + Lm;

    sigma = 1.0 - (Lm*Lm)/(Ls*Lr);

    kr = Lm/Lr;

    R_sigma = Rs + Rr*kr*kr;

    tau_r = Lr/Rr;
    tau_sigma = sigma*Ls/R_sigma;

    % Velocidad electrica del rotor.
    omega_r = p*wm;

    % ==============================================================
    % 3) Tabla de estados igual al selector actual
    % ==============================================================

    sel_a = [ ...
        1 3 2 1 2 3 ...
        1 1 1 1 1 1 1 ...
        2 2 2 2 2 2 2 ...
        3 3 3 3 3 3 3 ];

    sel_b = [ ...
        2 1 3 3 1 2 ...
        1 1 1 2 2 3 3 ...
        1 1 2 2 2 3 3 ...
        1 1 2 2 3 3 3 ];

    sel_c = [ ...
        3 2 1 2 3 1 ...
        1 2 3 1 2 1 3 ...
        1 2 1 2 3 2 3 ...
        1 3 2 3 1 2 3 ];

    idx = round(state_idx);

    if idx < 1
        idx = 1;
    elseif idx > 27
        idx = 27;
    end

    vin = [vA vB vC];

    src_a = sel_a(idx);
    src_b = sel_b(idx);
    src_c = sel_c(idx);

    % Tension de salida reconstruida segun estado aplicado
    va = vin(src_a);
    vb = vin(src_b);
    vc = vin(src_c);

    % abc -> alpha-beta
    vo_alpha = (2.0/3.0)*(va - 0.5*vb - 0.5*vc);
    vo_beta  = (1.0/sqrt(3.0))*(vb - vc);

    vo_a_out = vo_alpha;
    vo_b_out = vo_beta;

    % ==============================================================
    % 4) Corriente medida abc -> alpha-beta
    % ==============================================================

    i_alpha = (2.0/3.0)*(ia - 0.5*ib - 0.5*ic);
    i_beta  = (1.0/sqrt(3.0))*(ib - ic);
    
% ==============================================================
% Error de prediccion de la muestra anterior
% ==============================================================
%
% En el ciclo anterior se calculo ip_a_prev = i_alpha_pred(k).
% Ahora comparamos contra la corriente realmente medida i_alpha(k).

    if pred_valid
        err_a_out = i_alpha - ip_a_prev;
        err_b_out = i_beta  - ip_b_prev;
    else
        err_a_out = 0.0;
        err_b_out = 0.0;
        pred_valid = true;
    end

    err_abs_out = sqrt(err_a_out*err_a_out + err_b_out*err_b_out);

    % ==============================================================
    % 5) Estimador de flujo rotorico en marco estacionario alpha-beta
    % ==============================================================
    %
    % Modelo continuo, con omega_k = 0:
    %
    % d(psi_r)/dt =
    %   -psi_r/tau_r + j*omega_r*psi_r + (Lm/tau_r)*i_s
    %
    % Separado:
    %
    % dpsi_alpha = (-psi_alpha + Lm*i_alpha)/tau_r - omega_r*psi_beta
    % dpsi_beta  = (-psi_beta  + Lm*i_beta )/tau_r + omega_r*psi_alpha

    % Discretizacion exacta (ZOH sobre i), no Euler explicito:
    %   psi(k+1) = Phi*psi(k) + G*Lm*i(k)
    %   Phi = exp(A*Ts),  G = (Phi-1)/(A*tau_r),  A = -1/tau_r + j*omega_r
    ea = exp(-Ts_ctrl/tau_r);
    Phi_re = ea*cos(omega_r*Ts_ctrl);
    Phi_im = ea*sin(omega_r*Ts_ctrl);
    den_A = (1.0/tau_r)^2 + omega_r^2;
    G_re = (-(Phi_re - 1.0)/tau_r + Phi_im*omega_r)/(den_A*tau_r);
    G_im = (-Phi_im/tau_r - (Phi_re - 1.0)*omega_r)/(den_A*tau_r);

    psi_a_next = Phi_re*psi_a - Phi_im*psi_b + Lm*(G_re*i_alpha - G_im*i_beta);
    psi_b_next = Phi_im*psi_a + Phi_re*psi_b + Lm*(G_im*i_alpha + G_re*i_beta);

    % Proteccion defensiva: evita arrastrar NaN si algo se rompe.
    if ~isfinite(psi_a_next)
        psi_a_next = 0.0;
    end

    if ~isfinite(psi_b_next)
        psi_b_next = 0.0;
    end

    psi_a = psi_a_next;
    psi_b = psi_b_next;

    % ==============================================================
    % 6) Prediccion de corriente una muestra adelante
    % ==============================================================
    %
    % A partir de:
    %
    % i_s + tau_sigma*di_s/dt =
    %   (kr/R_sigma)*(1/tau_r - j*omega_r)*psi_r
    %   + v_s/R_sigma
    %
    % En componentes:
    %
    % (1/tau_r - j*omega_r)*(psi_a + j psi_b)
    % =
    % (psi_a/tau_r + omega_r*psi_b)
    % + j*(psi_b/tau_r - omega_r*psi_a)

    aux_a = psi_a/tau_r + omega_r*psi_b;
    aux_b = psi_b/tau_r - omega_r*psi_a;

    di_a = ( -i_alpha + (kr/R_sigma)*aux_a + vo_alpha/R_sigma )/tau_sigma;
    di_b = ( -i_beta  + (kr/R_sigma)*aux_b + vo_beta /R_sigma )/tau_sigma;

    ip_a_out = i_alpha + Ts_ctrl*di_a;
    ip_b_out = i_beta  + Ts_ctrl*di_b;
    
    % Guardar prediccion actual para compararla en el proximo ciclo
    ip_a_prev = ip_a_out;
    ip_b_prev = ip_b_out;
    

    % ==============================================================
    % 7) Salidas
    % ==============================================================

    psi_r_alpha = psi_a;
    psi_r_beta  = psi_b;

    psi_r_abs = sqrt(psi_a*psi_a + psi_b*psi_b);
    theta_psi = atan2(psi_b, psi_a);

    ip_alpha_pred = ip_a_out;
    ip_beta_pred  = ip_b_out;

    pred_err_alpha = err_a_out;
    pred_err_beta  = err_b_out;
    pred_err_abs   = err_abs_out;
end

== matlab function DMC_FCSMPC_IM_Physical_v6_3_L100_T1_EX28/MATLAB Function10 ==
  data: ia input; i_alpha output; ib input; ic input; i_beta output
function [i_alpha, i_beta] = abc_to_ab_monitor(ia,ib,ic)
%#codegen
    i_alpha = (2.0/3.0)*(ia - 0.5*ib - 0.5*ic);
    i_beta  = (1.0/sqrt(3.0))*(ib - ic);
end
